simulink model "full_order_observer_intro"  (R2025b)
settings: Solver=ode45  StartTime=0.0  StopTime=8  MaxStep=0.01  RelTol=1e-8  AbsTol=1e-10
settings Model: Creator=alosw  LastModifiedBy=alosw

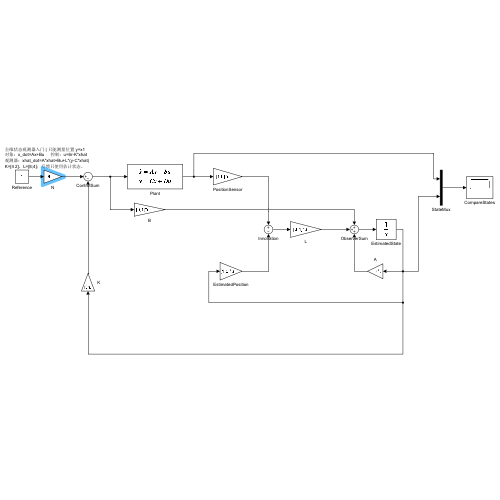
[thumbnail: Simulink's stored preview of the top-level diagram]
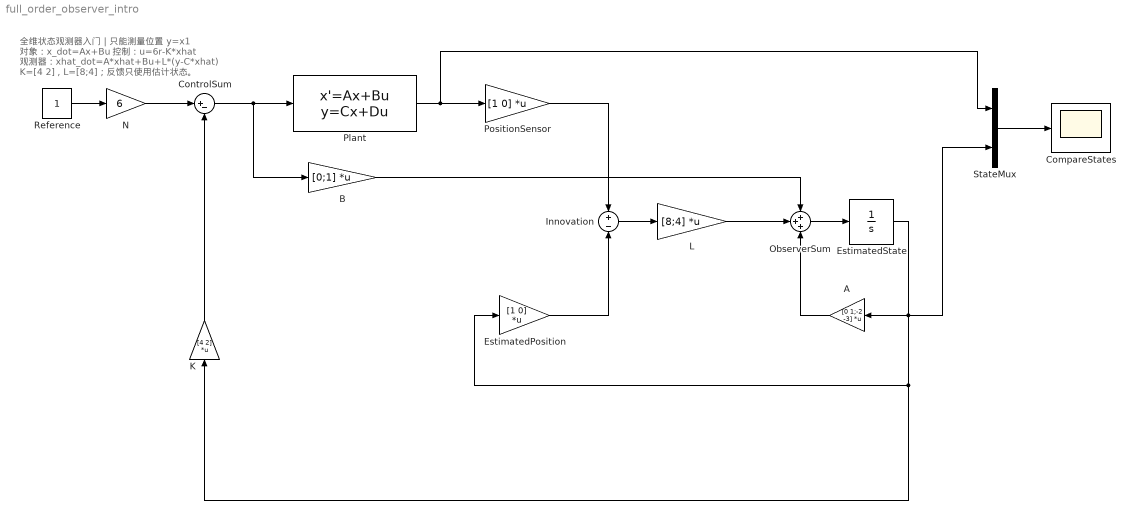
== system full_order_observer_intro ==
  note: 全维状态观测器入门 | 只能测量位置 y=x1
      | 对象：x_dot=Ax+Bu     控制：u=6r-K*xhat
      | 观测器：xhat_dot=A*xhat+Bu+L*(y-C*xhat)
      | K=[4 2]，L=[8;4]；反馈只使用估计状态。
  A : Gain  Gain=[0 1;-2 -3]  Multiplication=Matrix(K*u)
  B : Gain  Gain=[0;1]  Multiplication=Matrix(K*u)
  CompareStates : Scope
      settings: ActiveDisplayYMinimum=-0.40759477673564826  ActiveDisplayYMaximum=1.3512803888359621
  ControlSum : Sum  Inputs=|+-
  EstimatedPosition : Gain  Gain=[1 0]  Multiplication=Matrix(K*u)
  EstimatedState : Integrator  InitialCondition=[0;0]
  Innovation : Sum  Inputs=+-
  K : Gain  Gain=[4 2]  Multiplication=Matrix(K*u)
  L : Gain  Gain=[8;4]  Multiplication=Matrix(K*u)
  N : Gain  Gain=6
  ObserverSum : Sum  Inputs=+++
  Plant : StateSpace  A=[0 1;-2 -3]  B=[0;1]  C=eye(2)  D=zeros(2,1)  InitialCondition=[0.5;0]
  PositionSensor : Gain  Gain=[1 0]  Multiplication=Matrix(K*u)
  Reference : Constant
  StateMux : Mux  Inputs=2
  wires:
  Reference/1 -> N/1
  N/1 -> ControlSum/1
  ControlSum/1 -> B/1, Plant/1
  Plant/1 -> StateMux/1, PositionSensor/1
  PositionSensor/1 -> Innovation/1
  B/1 -> ObserverSum/1
  Innovation/1 -> L/1
  L/1 -> ObserverSum/2
  A/1 -> ObserverSum/3
  ObserverSum/1 -> EstimatedState/1
  EstimatedState/1 -> A/1, K/1, EstimatedPosition/1, StateMux/2
  EstimatedPosition/1 -> Innovation/2
  K/1 -> ControlSum/2
  StateMux/1 -> CompareStates/1
